simulink model "Simulation_cs_old"  (R2019a)
settings: Solver=ode5  StartTime=0.0  StopTime=inf  FixedStep=1/20  RelTol=1e-3
PreLoadFcn:
  | mbxruntime.callbacks.PreLoadFcn(bdroot);
PostLoadFcn:
  | mbxruntime.callbacks.PostLoadFcn(bdroot);
InitFcn:
  | mbxruntime.callbacks.InitFcn(bdroot);
StartFcn:
  | mbxruntime.callbacks.StartFcn(bdroot);
StopFcn:
  | mbxruntime.callbacks.StopFcn(bdroot);
model workspace: external: MAT-File .\Simulation_cs_hws.mat (data not in the file)
undefined symbols (not defined in the file or in its folder): DiscIntNeverNeededParam, InitImageOutputDir, mbxruntime, Simulation_cs_3ba1e87c6cdc7fd9, Simulation_cs_BMW_X5_SUV_1_Dynamics_Empty_STATE_BMW_X5_SUV_1_x0, Simulation_cs_BMW_X5_SUV_1_Dynamics_Empty_STATE_BMW_X5_SUV_1_y0, Simulation_cs_BMW_X5_SUV_1_Dynamics_Empty_STATE_BMW_X5_SUV_1_z0, Simulation_cs_dbe7801ee2d75073, Simulation_cs_f34d2d8469e03015
libraries: adeye_lib x45, robotlib x3, PreScanSimulinkLibrary x2, PreScanUsefulBlocks x1
(part 3 of 3)

== system Simulation_cs_old/PointCloudSensor_1 ==
  Sensor : S-Function  FunctionName=sfun_PCS  Parameters=mbxruntime.parameters.convert(sensorID), mbxruntime.parameters.convert(dataWidth), mbxruntime.parameters.convert(dataHeight), mbxruntime.parameters.convert(numChannels), mbxruntime.parameters.convert(dataType), mbxruntime.parameters.convert(timestep)  SFunctionDeploymentMode=off  EnableBusSupport=off  mask(PreScan Source Block: Point Cloud Sensor){sensorID=159, dataWidth=16, dataHeight=900, numChannels=4, dataType=0, timestep=1/20}
      mask prompts: sensorID "Sensor ID"; dataWidth "Data Width"; dataHeight "Data Height"; numChannels "Channel Count"; dataType "Data Type"; timestep "MATLAB timestep:"
      mask help: The Point Cloud Sensor provides XYZ positions relative to the sensor
      mask Help: eval('openHelp(6400)')
      mask Display: image(imread('PointCloudSensorSL.png'))
  PointCloudSensor_1 : Outport  Tag=outport/PointCloudInport  OutDataTypeStr=single  SampleTime=1/20
  wires:
  Sensor/1 -> PointCloudSensor_1/1

== system Simulation_cs_old/PointCloudSensor_2 ==
  Sensor : S-Function  FunctionName=sfun_PCS  Parameters=mbxruntime.parameters.convert(sensorID), mbxruntime.parameters.convert(dataWidth), mbxruntime.parameters.convert(dataHeight), mbxruntime.parameters.convert(numChannels), mbxruntime.parameters.convert(dataType), mbxruntime.parameters.convert(timestep)  SFunctionDeploymentMode=off  EnableBusSupport=off  mask(PreScan Source Block: Point Cloud Sensor){sensorID=160, dataWidth=16, dataHeight=900, numChannels=4, dataType=0, timestep=1/20}
      mask prompts: sensorID "Sensor ID"; dataWidth "Data Width"; dataHeight "Data Height"; numChannels "Channel Count"; dataType "Data Type"; timestep "MATLAB timestep:"
      mask help: The Point Cloud Sensor provides XYZ positions relative to the sensor
      mask Help: eval('openHelp(6400)')
      mask Display: image(imread('PointCloudSensorSL.png'))
  PointCloudSensor_2 : Outport  Tag=outport/PointCloudInport  OutDataTypeStr=single  SampleTime=1/20
  wires:
  Sensor/1 -> PointCloudSensor_2/1

== system Simulation_cs_old/PointCloudSensor_3 ==
  Sensor : S-Function  FunctionName=sfun_PCS  Parameters=mbxruntime.parameters.convert(sensorID), mbxruntime.parameters.convert(dataWidth), mbxruntime.parameters.convert(dataHeight), mbxruntime.parameters.convert(numChannels), mbxruntime.parameters.convert(dataType), mbxruntime.parameters.convert(timestep)  SFunctionDeploymentMode=off  EnableBusSupport=off  mask(PreScan Source Block: Point Cloud Sensor){sensorID=161, dataWidth=16, dataHeight=900, numChannels=4, dataType=0, timestep=1/20}
      mask prompts: sensorID "Sensor ID"; dataWidth "Data Width"; dataHeight "Data Height"; numChannels "Channel Count"; dataType "Data Type"; timestep "MATLAB timestep:"
      mask help: The Point Cloud Sensor provides XYZ positions relative to the sensor
      mask Help: eval('openHelp(6400)')
      mask Display: image(imread('PointCloudSensorSL.png'))
  PointCloudSensor_3 : Outport  Tag=outport/PointCloudInport  OutDataTypeStr=single  SampleTime=1/20
  wires:
  Sensor/1 -> PointCloudSensor_3/1

== system Simulation_cs_old/PointCloudSensor_4 ==
  Sensor : S-Function  FunctionName=sfun_PCS  Parameters=mbxruntime.parameters.convert(sensorID), mbxruntime.parameters.convert(dataWidth), mbxruntime.parameters.convert(dataHeight), mbxruntime.parameters.convert(numChannels), mbxruntime.parameters.convert(dataType), mbxruntime.parameters.convert(timestep)  SFunctionDeploymentMode=off  EnableBusSupport=off  mask(PreScan Source Block: Point Cloud Sensor){sensorID=162, dataWidth=16, dataHeight=900, numChannels=4, dataType=0, timestep=1/20}
      mask prompts: sensorID "Sensor ID"; dataWidth "Data Width"; dataHeight "Data Height"; numChannels "Channel Count"; dataType "Data Type"; timestep "MATLAB timestep:"
      mask help: The Point Cloud Sensor provides XYZ positions relative to the sensor
      mask Help: eval('openHelp(6400)')
      mask Display: image(imread('PointCloudSensorSL.png'))
  PointCloudSensor_4 : Outport  Tag=outport/PointCloudInport  OutDataTypeStr=single  SampleTime=1/20
  wires:
  Sensor/1 -> PointCloudSensor_4/1

== system Simulation_cs_old/PreScanTerminator ==
  Terminator : Terminator
  sfun_Terminator : S-Function  FunctionName=sfun_Terminator  Parameters=SampleTime  SFunctionDeploymentMode=off  EnableBusSupport=off  mask(Legacy Function){SFunctionSpec=void prescan_terminator_outputFcn(void ** work1, PRESCAN_TERMINATORDATA y1[1]), SampleTime=TimeStep, ShowSpec=on}
      mask prompts: SampleTime "Sample time (-1 for inherited):"; ShowSpec "Display function specification"
      mask help:
      | This block allows you to call the legacy functions specified by the following Legacy Code Tool definition:
      | def.SFunctionName = 'sfun_Terminator';
      | def.OutputFcnSpec = 'void prescan_terminator_outputFcn(void ** work1, PRESCAN_TERMINATORDATA y1[1])';
      | def.StartFcnSpec = 'void prescan_terminator_startFcn(void ** work1)';
      | def.TerminateFcnSpec = 'void prescan_terminator_terminateFcn(void ** work1)';
      | def.HeaderFiles = {'prescan_terminator_data.h'};
      | def.HostLibFiles = {'sensorinterfaced.lib'};
      | def.IncPaths = {'src', 'C:\prescandev\vislibrary\vis\..\pimp\include\sensors\InterfaceRTW'};
      | def.SrcPaths = {'src'};
      | def.LibPaths = {'C:\\prescandev\\vislibrary_build\lib'};
      | def.SampleTime = 'parameterized';
      | def.Options.language = 'C';
      mask Help: <p>This block was generated automatically by the Legacy Code Tool. For detailed help on this tool, call<a href="matlab:legacy_code('help')"> legacy_code('help')</a>.</p>
      mask Callback ShowSpec:
      | if strcmp(get_param(gcbh, 'ShowSpec'), 'on')
      |   set_param(gcbh, 'MaskDisplay', sprintf('fprintf(''%s'');', get_param(gcbh, 'SFunctionSpec')));
      | else
      |   set_param(gcbh, 'MaskDisplay', sprintf('fprintf(''%s'');', get_param(gcbh, 'FunctionName')));
      | end
      mask Display: fprintf('void prescan_terminator_outputFcn(void ** work1, PRESCAN_TERMINATORDATA y1[1])');
  wires:
  sfun_Terminator/1 -> Terminator/1

== system Simulation_cs_old/Radar_1 ==
  Sensor : S-Function  FunctionName=sfun_Radar  Parameters=mbxruntime.parameters.convert(sensorID), mbxruntime.parameters.convert(detectableObjects), mbxruntime.parameters.convert(timestep)  SFunctionDeploymentMode=off  EnableBusSupport=off  mask(PreScan Source Block: Radar Sensor){sensorID=165, detectableObjects=7, timestep=1/20}
      mask prompts: sensorID "Sensor ID"; detectableObjects "Max detectable objects:"; timestep "MATLAB timestep:"
      mask help:
      | The Radar Sensor is a detailed sensor based on a physical radar
      | model that includes Antenna GAIN Maps (AGM) and atmospheric
      | attenuation.
      |
      | For more information, please click Help.
      mask Help: eval('openHelp(1464)')
      mask Display: image(imread('Radar.png'))
  Radar_1 : Outport  Tag=outport/Radar  OutDataTypeStr=Bus: PRESCAN_SCANNERSENSOR_MESSAGE  PortDimensions=7  SampleTime=1/20
  wires:
  Sensor/1 -> Radar_1/1

== system Simulation_cs_old/SELF_BMW_X5_SUV_1 ==
  Sensor : S-Function  FunctionName=sfun_SelfSensor  Parameters=mbxruntime.parameters.convert(UniqueID), mbxruntime.parameters.convert(TimeStep)  SFunctionDeploymentMode=off  EnableBusSupport=off  mask(PreScan Source Block: SELF){UniqueID=158, TimeStep=1/20}
      mask prompts: UniqueID "Auto-Assigned: Unique ID"; TimeStep "Auto-Assigned: Upload Period [s]"
      mask help:
      | The SELF port shows (state) information of the actor itself. The outputs are position in the experiment's axis system and the GPS coordinates, and the object's absolute velocity and compass heading.
      |
      | For more information, please click Help.
      mask Help: eval('openHelp(462)')
      mask Display: image(imread('GPS.png'))
  SELF_BMW_X5_SUV_1 : Outport  Tag=outport/SelfPort  OutDataTypeStr=Bus: PRESCAN_SELFSENSORDATA  PortDimensions=1  SampleTime=1/20
  wires:
  Sensor/1 -> SELF_BMW_X5_SUV_1/1

== system Simulation_cs_old/STATE_BMW_X5_SUV_1_bus ==
  STATE_BMW_X5_SUV_1_bus : Inport  Tag=inport/StatePort  OutDataTypeStr=Bus: PRESCAN_STATEACTUATORDATA  PortDimensions=1  SampleTime=1/20  BusOutputAsStruct=on
  Actuator : S-Function  FunctionName=sfun_StateActuator  Parameters=mbxruntime.parameters.convert(UniqueID), mbxruntime.parameters.convert(TimeStep)  SFunctionDeploymentMode=off  EnableBusSupport=off  mask(PreScan Sink Block: State){UniqueID=158, TimeStep=1/20}
      mask prompts: UniqueID "Auto-Assigned: Unique ID"; TimeStep "Auto-Assigned: Upload Period [s]"
      mask help:
      | The Actor State contains a vector signal of size (9x1), containing the following signals:
      |
      | -  Position    	(x,y,z)             	[m]
      | -  Velocity    	(vx,vy,vz)         	[m/s]
      | -  Angles       	(Roll, Pitch, Yaw)	[rad]
      |
      | The Actor state is defined in the global axis system.
      | The state is superponed on the Initial position defined in the GUI.
      |
      | For more information, please click Help.
      mask Help: eval('openHelp(222)')
      mask Display: image(imread('State.png'))
  wires:
  STATE_BMW_X5_SUV_1_bus/1 -> Actuator/1

== system Simulation_cs_old/ScenarioEngine ==
  Clock : Clock
  sfun_ScenarioEngine : S-Function  FunctionName=sfun_ScenarioEngine  Parameters=TimeStep  SFunctionDeploymentMode=off  EnableBusSupport=off
  wires:
  Clock/1 -> sfun_ScenarioEngine/1

== system Simulation_cs_old/Synchronizer ==
  Bus Selector1 : BusSelector  OutputSignals=FederateStopped
  Stop Simulation : Stop
  sfun_Synchronizer : S-Function  FunctionName=sfun_Synchronizer  Parameters=SampleTime  SFunctionDeploymentMode=off  EnableBusSupport=off  mask(Legacy Function){SFunctionSpec=void prescan_synchronizer_outputFcn(void ** work1, PRESCAN_SYNCHRONIZEDATA y1[1]), SampleTime=TimeStep, ShowSpec=on}
      mask prompts: SampleTime "Sample time (-1 for inherited):"; ShowSpec "Display function specification"
      mask help:
      | This block allows you to call the legacy functions specified by the following Legacy Code Tool definition:
      | def.SFunctionName = 'sfun_Synchronizer';
      | def.OutputFcnSpec = 'void prescan_synchronizer_outputFcn(void ** work1, PRESCAN_TIMESTAMPDATA u1[1], PRESCAN_SYNCHRONIZEDATA y1[1])';
      | def.StartFcnSpec = 'void prescan_synchronizer_startFcn(void ** work1)';
      | def.TerminateFcnSpec = 'void prescan_synchronizer_terminateFcn(void ** work1)';
      | def.HeaderFiles = {'prescan_synchronizer_data.h'};
      | def.HostLibFiles = {'sensorinterfaced.lib'};
      | def.IncPaths = {'src', 'C:\prescandev\vislibrary\vis\..\pimp\include\sensors\InterfaceRTW'};
      | def.SrcPaths = {'src'};
      | def.LibPaths = {'C:\\prescandev\\vislibrary_build\lib'};
      | def.SampleTime = 'parameterized';
      | def.Options.language = 'C';
      mask Help: <p>This block was generated automatically by the Legacy Code Tool. For detailed help on this tool, call<a href="matlab:legacy_code('help')"> legacy_code('help')</a>.</p>
      mask Callback ShowSpec:
      | if strcmp(get_param(gcbh, 'ShowSpec'), 'on')
      |   set_param(gcbh, 'MaskDisplay', sprintf('fprintf(''%s'');', get_param(gcbh, 'SFunctionSpec')));
      | else
      |   set_param(gcbh, 'MaskDisplay', sprintf('fprintf(''%s'');', get_param(gcbh, 'FunctionName')));
      | end
      mask Display: fprintf('void prescan_synchronizer_outputFcn(void ** work1, PRESCAN_SYNCHRONIZEDATA y1[1])');
  wires:
  sfun_Synchronizer/1 -> Bus Selector1/1
  Bus Selector1/1 -> Stop Simulation/1  "<FederateStopped>"

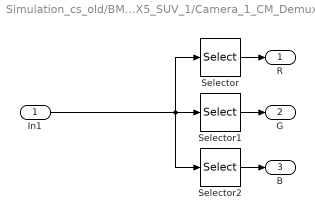
== system Simulation_cs_old/BMW_X5_SUV_1/Camera_1_CM_Demux ==
  In1 : Inport
  Selector : Selector  NumberOfDimensions=2  InputPortWidth=3  IndexOptions=Index vector (dialog),Index vector (dialog)  Indices=-1,1:hres  OutputSizes=1,1
  Selector1 : Selector  NumberOfDimensions=2  InputPortWidth=3  IndexOptions=Index vector (dialog),Index vector (dialog)  Indices=-1,hres+1:hres*2  OutputSizes=1,1
  Selector2 : Selector  NumberOfDimensions=2  InputPortWidth=3  IndexOptions=Index vector (dialog),Index vector (dialog)  Indices=-1,hres*2+1:hres*3  OutputSizes=1,1
  R : Outport
  G : Outport  Port=2
  B : Outport  Port=3
  wires:
  In1/1 -> Selector1/1, Selector/1, Selector2/1
  Selector/1 -> R/1
  Selector1/1 -> G/1
  Selector2/1 -> B/1

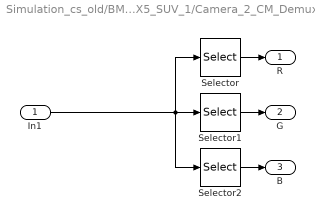
== system Simulation_cs_old/BMW_X5_SUV_1/Camera_2_CM_Demux ==
  In1 : Inport
  Selector : Selector  NumberOfDimensions=2  InputPortWidth=3  IndexOptions=Index vector (dialog),Index vector (dialog)  Indices=-1,1:hres  OutputSizes=1,1
  Selector1 : Selector  NumberOfDimensions=2  InputPortWidth=3  IndexOptions=Index vector (dialog),Index vector (dialog)  Indices=-1,hres+1:hres*2  OutputSizes=1,1
  Selector2 : Selector  NumberOfDimensions=2  InputPortWidth=3  IndexOptions=Index vector (dialog),Index vector (dialog)  Indices=-1,hres*2+1:hres*3  OutputSizes=1,1
  R : Outport
  G : Outport  Port=2
  B : Outport  Port=3
  wires:
  In1/1 -> Selector1/1, Selector/1, Selector2/1
  Selector/1 -> R/1
  Selector1/1 -> G/1
  Selector2/1 -> B/1

== system Simulation_cs_old/BMW_X5_SUV_1/Camera_tl_CM_Demux ==
  In1 : Inport
  Selector : Selector  NumberOfDimensions=2  InputPortWidth=3  IndexOptions=Index vector (dialog),Index vector (dialog)  Indices=-1,1:hres  OutputSizes=1,1
  Selector1 : Selector  NumberOfDimensions=2  InputPortWidth=3  IndexOptions=Index vector (dialog),Index vector (dialog)  Indices=-1,hres+1:hres*2  OutputSizes=1,1
  Selector2 : Selector  NumberOfDimensions=2  InputPortWidth=3  IndexOptions=Index vector (dialog),Index vector (dialog)  Indices=-1,hres*2+1:hres*3  OutputSizes=1,1
  R : Outport
  G : Outport  Port=2
  B : Outport  Port=3
  wires:
  In1/1 -> Selector1/1, Selector/1, Selector2/1
  Selector/1 -> R/1
  Selector1/1 -> G/1
  Selector2/1 -> B/1

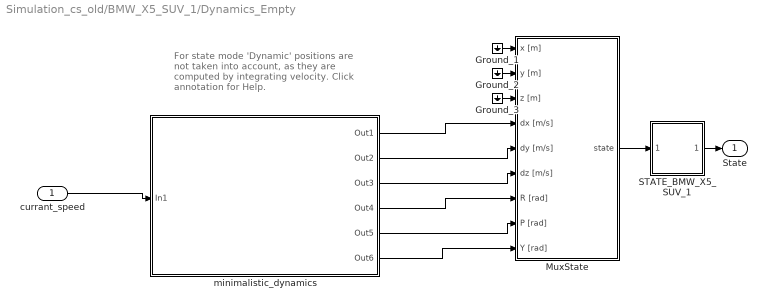
== system Simulation_cs_old/BMW_X5_SUV_1/Dynamics_Empty ==
  note: For state mode 'Dynamic' positions
      | are not taken into account, as they
      | are computed by integrating velocity.
      | Click annotation for Help.
  currant_speed : Inport
  Ground_1 : Ground
  Ground_2 : Ground
  Ground_3 : Ground
  MuxState : Subsystem  Tag=mux/State  mask(Empty Dynamics State Block){positioningmode=off, TimeStep=1/20}
      mask prompts: positioningmode "Positioning Mode"; TimeStep "Auto Assigned: Time Step [s]"
      mask help:
      | Build the state of an actor based on user input.
      | The user can either use positioning mode or dynamics mode.
      | - When using positioning mode the position and orientation of the actor are set directly based on the input. Expected input is relative to the initial position and orientation of the actor. It's also possible to specify the velocity of the actor, though this input isn't used, only passed on.
      | - When using dynamics mode the position input is ignored. Expected input is velocity and orientation. The velocity is relative the current orientation of the actor, while orientation is relative to its initial orientation. The position of the actor is calculated based on the velocity and orientation given.
      settings: DeleteFcn=PreScanBlockDeleteFcn;
  STATE_BMW_X5_SUV_1 : Subsystem  Tag=mux/StatePort  Priority=0  LoadFcn=load PrescanStateActuatorData  mask(PreScan Sink Block: State){x0=Simulation_cs_BMW_X5_SUV_1_Dynamics_Empty_STATE_BMW_X5_SUV_1_x0, y0=Simulation_cs_BMW_X5_SUV_1_Dynamics_Empty_STATE_BMW_X5_SUV_1_y0, z0=Simulation_cs_BMW_X5_SUV_1_Dynamics_Empty_STATE_BMW_X5_SUV_1_z0, Roll0=Simulation_cs_dbe7801ee2d75073, Pitch0=Simulation_cs_3ba1e87c6cdc7fd9, Yaw0=Simulation_cs_f34d2d8469e03015, TimeStep=1/20}
      mask prompts: x0 "Ini x-position VEHICLE wrt GLOBAL axis system [m]"; y0 "Ini y-position VEHICLE wrt GLOBAL axis system [m]"; z0 "Ini z-position VEHICLE wrt GLOBAL axis system [m]"; Roll0 "Ini roll-angle BODY wrt VEHICLE axis system [deg]"; Pitch0 "Ini pitch-angle BODY wrt VEHICLE axis system [deg]"; Yaw0 "Ini yaw-angle VEHICLE wrt GLOBAL axis system [deg]"; TimeStep "Auto-Assigned: Upload Period [s]"
      mask help:
      | The Actor State contains a vector signal of size (9x1), containing the following signals:
      |
      | -  Position                  (x,y,z)                                     [m]
      | -  Velocity                  (vx,vy,vz)                               [m/s]
      | -  Angles                    (Roll, Pitch, Yaw)                   [rad]
      |
      | The Actor state is defined in the global axis system.
      | The state is superponed on the Initial position defined in the GUI.
      |
      | For more information, please click Help.
      settings: DeleteFcn=PreScanBlockDeleteFcn;
      mask Help: eval('openHelp(222)')
      mask Display: image(imread('State.png'))
  minimalistic_dynamics : Subsystem  AncestorBlock=adeye_lib/minimalistic_dynamics
      mask Display:
      | fprintf('Minimalistic Dynamics\n\n')
      | 
      | port_label('input',1,'velocity[m/s]')
      | 
      | port_label('output',1,'dx [m/s]')
      | port_label('output',2,'dy [m/s]')
      | port_label('output',3,'dz [m/s]')
      | port_label('output',4,'R [rad]')
      | port_label('output',5,'P [rad]')
      | port_label('output',6,'Y [rad]')
  State : Outport  Tag=outport/StateOutport  SampleTime=1/20
  wires:
  minimalistic_dynamics/1(Out1) -> MuxState/4(dx [m/s])
  minimalistic_dynamics/2(Out2) -> MuxState/5(dy [m/s])
  minimalistic_dynamics/3(Out3) -> MuxState/6(dz [m/s])
  minimalistic_dynamics/4(Out4) -> MuxState/7(R [rad])
  minimalistic_dynamics/5(Out5) -> MuxState/8(P [rad])
  minimalistic_dynamics/6(Out6) -> MuxState/9(Y [rad])
  currant_speed/1 -> minimalistic_dynamics/1(In1)
  MuxState/1(state) -> STATE_BMW_X5_SUV_1/1(State)
  STATE_BMW_X5_SUV_1/1(StateBus) -> State/1
  Ground_1/1 -> MuxState/1(x [m])
  Ground_2/1 -> MuxState/2(y [m])
  Ground_3/1 -> MuxState/3(z [m])

== system Simulation_cs_old/BMW_X5_SUV_1/PointCloudSensor_1_Angles_Demux ==
  In2 : Inport
  Selector : Selector  NumberOfDimensions=2  InputPortWidth=3  IndexOptions=Index vector (dialog),Index vector (dialog)  Indices=-1,offset+1:(offset+hres)  OutputSizes=1,1
  Selector1 : Selector  NumberOfDimensions=2  InputPortWidth=3  IndexOptions=Index vector (dialog),Index vector (dialog)  Indices=-1,(offset+hres+1):(offset+2*hres)  OutputSizes=1,1
  Theta : Outport
  Phi : Outport  Port=2
  wires:
  Selector1/1 -> Phi/1
  Selector/1 -> Theta/1
  In2/1 -> Selector/1, Selector1/1

== system Simulation_cs_old/BMW_X5_SUV_1/PointCloudSensor_1_Intensity_Demux ==
  In1 : Inport
  Selector3 : Selector  NumberOfDimensions=2  InputPortWidth=3  IndexOptions=Index vector (dialog),Index vector (dialog)  Indices=-1,offset+1:(offset+hres)  OutputSizes=1,1
  Intensity : Outport
  wires:
  Selector3/1 -> Intensity/1
  In1/1 -> Selector3/1

== system Simulation_cs_old/BMW_X5_SUV_1/PointCloudSensor_1_Range_Demux ==
  In1 : Inport
  Selector : Selector  NumberOfDimensions=2  InputPortWidth=3  IndexOptions=Index vector (dialog),Index vector (dialog)  Indices=-1,offset+1:(offset+hres)  OutputSizes=1,1
  Range : Outport
  wires:
  Selector/1 -> Range/1
  In1/1 -> Selector/1

== system Simulation_cs_old/BMW_X5_SUV_1/PointCloudSensor_2_Angles_Demux ==
  In2 : Inport
  Selector : Selector  NumberOfDimensions=2  InputPortWidth=3  IndexOptions=Index vector (dialog),Index vector (dialog)  Indices=-1,offset+1:(offset+hres)  OutputSizes=1,1
  Selector1 : Selector  NumberOfDimensions=2  InputPortWidth=3  IndexOptions=Index vector (dialog),Index vector (dialog)  Indices=-1,(offset+hres+1):(offset+2*hres)  OutputSizes=1,1
  Theta : Outport
  Phi : Outport  Port=2
  wires:
  Selector1/1 -> Phi/1
  Selector/1 -> Theta/1
  In2/1 -> Selector/1, Selector1/1

== system Simulation_cs_old/BMW_X5_SUV_1/PointCloudSensor_2_Intensity_Demux ==
  In1 : Inport
  Selector3 : Selector  NumberOfDimensions=2  InputPortWidth=3  IndexOptions=Index vector (dialog),Index vector (dialog)  Indices=-1,offset+1:(offset+hres)  OutputSizes=1,1
  Intensity : Outport
  wires:
  Selector3/1 -> Intensity/1
  In1/1 -> Selector3/1

== system Simulation_cs_old/BMW_X5_SUV_1/PointCloudSensor_2_Range_Demux ==
  In1 : Inport
  Selector : Selector  NumberOfDimensions=2  InputPortWidth=3  IndexOptions=Index vector (dialog),Index vector (dialog)  Indices=-1,offset+1:(offset+hres)  OutputSizes=1,1
  Range : Outport
  wires:
  Selector/1 -> Range/1
  In1/1 -> Selector/1

== system Simulation_cs_old/BMW_X5_SUV_1/PointCloudSensor_3_Angles_Demux ==
  In2 : Inport
  Selector : Selector  NumberOfDimensions=2  InputPortWidth=3  IndexOptions=Index vector (dialog),Index vector (dialog)  Indices=-1,offset+1:(offset+hres)  OutputSizes=1,1
  Selector1 : Selector  NumberOfDimensions=2  InputPortWidth=3  IndexOptions=Index vector (dialog),Index vector (dialog)  Indices=-1,(offset+hres+1):(offset+2*hres)  OutputSizes=1,1
  Theta : Outport
  Phi : Outport  Port=2
  wires:
  Selector1/1 -> Phi/1
  Selector/1 -> Theta/1
  In2/1 -> Selector/1, Selector1/1

== system Simulation_cs_old/BMW_X5_SUV_1/PointCloudSensor_3_Intensity_Demux ==
  In1 : Inport
  Selector3 : Selector  NumberOfDimensions=2  InputPortWidth=3  IndexOptions=Index vector (dialog),Index vector (dialog)  Indices=-1,offset+1:(offset+hres)  OutputSizes=1,1
  Intensity : Outport
  wires:
  Selector3/1 -> Intensity/1
  In1/1 -> Selector3/1

== system Simulation_cs_old/BMW_X5_SUV_1/PointCloudSensor_3_Range_Demux ==
  In1 : Inport
  Selector : Selector  NumberOfDimensions=2  InputPortWidth=3  IndexOptions=Index vector (dialog),Index vector (dialog)  Indices=-1,offset+1:(offset+hres)  OutputSizes=1,1
  Range : Outport
  wires:
  Selector/1 -> Range/1
  In1/1 -> Selector/1

== system Simulation_cs_old/BMW_X5_SUV_1/PointCloudSensor_4_Angles_Demux ==
  In2 : Inport
  Selector : Selector  NumberOfDimensions=2  InputPortWidth=3  IndexOptions=Index vector (dialog),Index vector (dialog)  Indices=-1,offset+1:(offset+hres)  OutputSizes=1,1
  Selector1 : Selector  NumberOfDimensions=2  InputPortWidth=3  IndexOptions=Index vector (dialog),Index vector (dialog)  Indices=-1,(offset+hres+1):(offset+2*hres)  OutputSizes=1,1
  Theta : Outport
  Phi : Outport  Port=2
  wires:
  Selector1/1 -> Phi/1
  Selector/1 -> Theta/1
  In2/1 -> Selector/1, Selector1/1

== system Simulation_cs_old/BMW_X5_SUV_1/PointCloudSensor_4_Intensity_Demux ==
  In1 : Inport
  Selector3 : Selector  NumberOfDimensions=2  InputPortWidth=3  IndexOptions=Index vector (dialog),Index vector (dialog)  Indices=-1,offset+1:(offset+hres)  OutputSizes=1,1
  Intensity : Outport
  wires:
  Selector3/1 -> Intensity/1
  In1/1 -> Selector3/1

== system Simulation_cs_old/BMW_X5_SUV_1/PointCloudSensor_4_Range_Demux ==
  In1 : Inport
  Selector : Selector  NumberOfDimensions=2  InputPortWidth=3  IndexOptions=Index vector (dialog),Index vector (dialog)  Indices=-1,offset+1:(offset+hres)  OutputSizes=1,1
  Range : Outport
  wires:
  Selector/1 -> Range/1
  In1/1 -> Selector/1

== system Simulation_cs_old/BMW_X5_SUV_1/Radar_1_Demux ==
  Radar : Inport
  Bus Selector1 : BusSelector  OutputSignals=ActiveBeamID[-],Range[m],DopplerVelocity[ms-1],DopplerVelocityX[ms-1],DopplerVelocityY[ms-1],DopplerVelocityZ[ms-1],Theta[deg],Phi[deg],TargetID[-],TargetTypeID[-],EnergyLoss[dB],Alpha[deg],Beta[deg]  OutputAsBus=on
  ScannerSensorLegacyBusConversion : PreScanUsefulBlocks/ScannerSensorLegacyBusConversion  MAXMESSAGES=MAXMESSAGES
  Radar Data : Outport
  Timestamp : Outport  Port=2
  wires:
  ScannerSensorLegacyBusConversion/2 -> Timestamp/1
  Bus Selector1/1 -> Radar Data/1
  ScannerSensorLegacyBusConversion/1 -> Bus Selector1/1
  Radar/1 -> ScannerSensorLegacyBusConversion/1

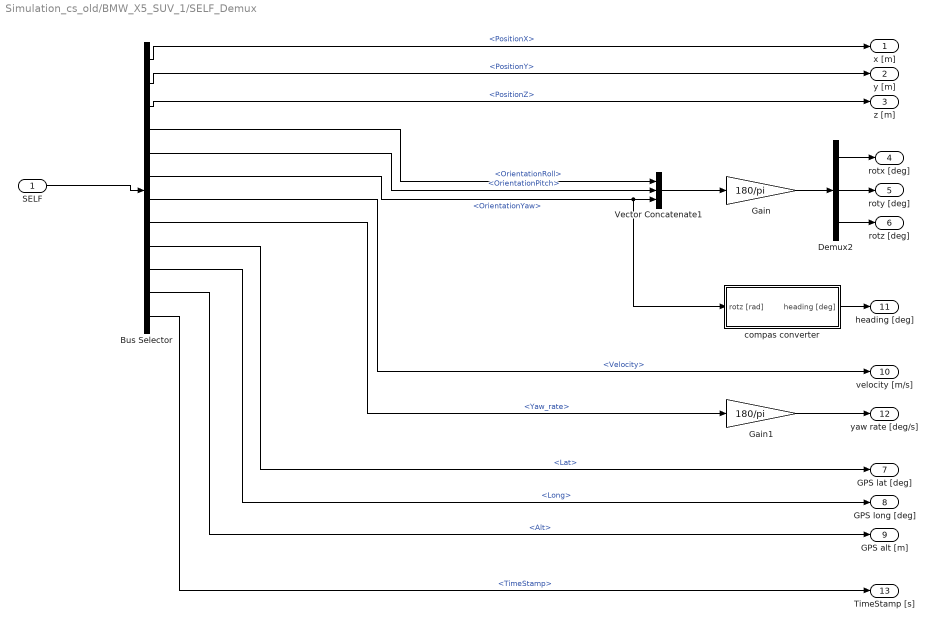
== system Simulation_cs_old/BMW_X5_SUV_1/SELF_Demux ==
  SELF : Inport  OutDataTypeStr=Bus: PRESCAN_SELFSENSORDATA
  Bus Selector : BusSelector  OutputSignals=PositionX,PositionY,PositionZ,OrientationRoll,OrientationPitch,OrientationYaw,Velocity,Yaw_rate,Lat,Long,Alt,TimeStamp
  Demux2 : Demux  Outputs=3
  Gain : Gain  Gain=180/pi
  Gain1 : Gain  Gain=180/pi
  Vector Concatenate1 : Concatenate  NumInputs=3
  compas converter : Subsystem
  x [m] : Outport
  y [m] : Outport  Port=2
  z [m] : Outport  Port=3
  rotx [deg] : Outport  Port=4
  roty [deg] : Outport  Port=5
  rotz [deg] : Outport  Port=6
  GPS lat [deg] : Outport  Port=7
  GPS long [deg] : Outport  Port=8
  GPS alt [m] : Outport  Port=9
  velocity [m/s] : Outport  Port=10
  heading [deg] : Outport  Port=11
  yaw rate [deg/s] : Outport  Port=12
  TimeStamp [s] : Outport  Port=13
  wires:
  Bus Selector/12 -> TimeStamp [s]/1  "<TimeStamp>"
  Bus Selector/11 -> GPS alt [m]/1  "<Alt>"
  Bus Selector/10 -> GPS long [deg]/1  "<Long>"
  Bus Selector/9 -> GPS lat [deg]/1  "<Lat>"
  Bus Selector/8 -> Gain1/1  "<Yaw_rate>"
  Bus Selector/7 -> velocity [m/s]/1  "<Velocity>"
  Bus Selector/6 -> compas converter/1(rotz [rad]), Vector Concatenate1/3  "<OrientationYaw>"
  Bus Selector/5 -> Vector Concatenate1/2  "<OrientationPitch>"
  Bus Selector/4 -> Vector Concatenate1/1  "<OrientationRoll>"
  Vector Concatenate1/1 -> Gain/1
  Bus Selector/3 -> z [m]/1  "<PositionZ>"
  Bus Selector/2 -> y [m]/1  "<PositionY>"
  Bus Selector/1 -> x [m]/1  "<PositionX>"
  SELF/1 -> Bus Selector/1
  Gain/1 -> Demux2/1
  Demux2/1 -> rotx [deg]/1
  Demux2/2 -> roty [deg]/1
  Demux2/3 -> rotz [deg]/1
  compas converter/1(heading [deg]) -> heading [deg]/1
  Gain1/1 -> yaw rate [deg/s]/1

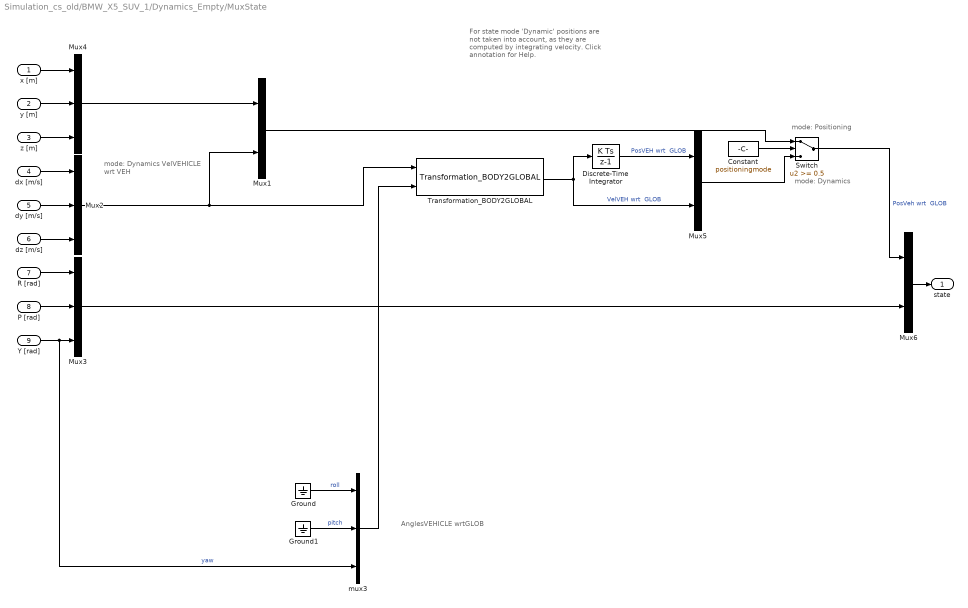
== system Simulation_cs_old/BMW_X5_SUV_1/Dynamics_Empty/MuxState ==
  note: mode: Dynamics
  note: mode: Positioning
  note: mode: Dynamics
      | VelVEHICLE
      | wrt VEH
  note: AnglesVEHICLE
      | wrtGLOB
  note: For state mode 'Dynamic' positions
      | are not taken into account, as they
      | are computed by integrating velocity.
      | Click annotation for Help.
  x [m] : Inport  SampleTime=TimeStep
  y [m] : Inport  Port=2  SampleTime=TimeStep
  z [m] : Inport  Port=3  SampleTime=TimeStep
  dx [m/s] : Inport  Port=4  SampleTime=TimeStep
  dy [m/s] : Inport  Port=5  SampleTime=TimeStep
  dz [m/s] : Inport  Port=6  SampleTime=TimeStep
  R [rad] : Inport  Port=7  SampleTime=TimeStep
  P [rad] : Inport  Port=8  SampleTime=TimeStep
  Y [rad] : Inport  Port=9  SampleTime=TimeStep
  Constant : Constant  DisableCoverage=on  Value=positioningmode
  Discrete-Time Integrator : DiscreteIntegrator  SampleTime=TimeStep  ICPrevOutput=DiscIntNeverNeededParam  ICPrevScaledInput=DiscIntNeverNeededParam
  Ground : Ground
  Ground1 : Ground
  Mux1 : Mux  Inputs=[3 3]
  Mux2 : Mux  Inputs=3
  Mux3 : Mux  Inputs=3
  Mux4 : Mux  Inputs=3
  Mux5 : Mux  Inputs=[3 3]
  Mux6 : Mux  Inputs=[6 3]
  Switch : Switch  Threshold=0.5
  Transformation_BODY2GLOBAL : PreScanSimulinkLibrary/Simple_Vehicle_Dynamics/Chassis/MuxDynState/Transformation_BODY2GLOBAL  SystemSampleTime=-1
  mux3 : Mux  Inputs=3
  state : Outport
  wires:
  Constant/1 -> Switch/2
  Mux6/1 -> state/1
  Mux4/1 -> Mux1/1
  Mux5/1 -> Switch/3
  Mux1/1 -> Switch/1
  Switch/1 -> Mux6/1  "PosVeh wrt  GLOB"
  P [rad]/1 -> Mux3/2
  R [rad]/1 -> Mux3/1
  dz [m/s]/1 -> Mux2/3
  dy [m/s]/1 -> Mux2/2
  dx [m/s]/1 -> Mux2/1
  z [m]/1 -> Mux4/3
  y [m]/1 -> Mux4/2
  x [m]/1 -> Mux4/1
  Ground1/1 -> mux3/2  "pitch"
  Y [rad]/1 -> mux3/3, Mux3/3  "yaw"
  Mux3/1 -> Mux6/2
  Transformation_BODY2GLOBAL/1 -> Discrete-Time Integrator/1, Mux5/2  "VelVEH wrt  GLOB"
  mux3/1 -> Transformation_BODY2GLOBAL/2
  Ground/1 -> mux3/1  "roll"
  Mux2/1 -> Mux1/2, Transformation_BODY2GLOBAL/1
  Discrete-Time Integrator/1 -> Mux5/1  "PosVEH wrt  GLOB"

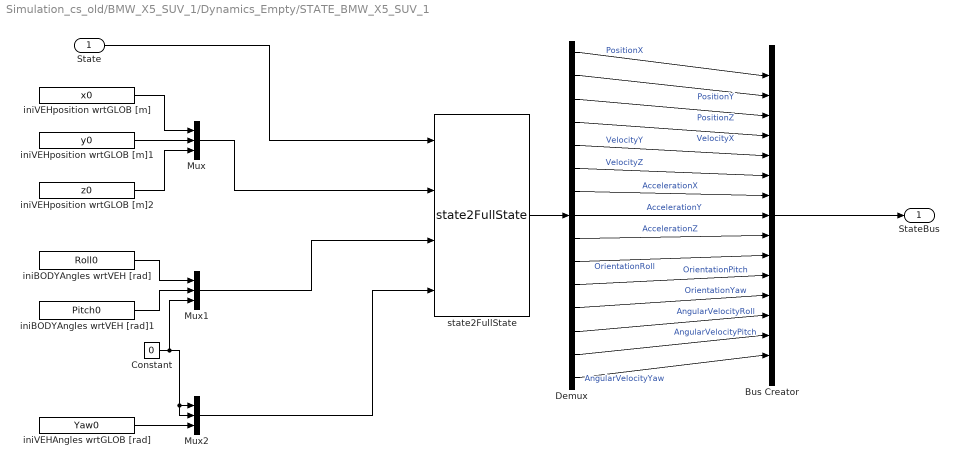
== system Simulation_cs_old/BMW_X5_SUV_1/Dynamics_Empty/STATE_BMW_X5_SUV_1 ==
  State : Inport  SampleTime=TimeStep
  Bus Creator : BusCreator  Inputs=15  OutDataTypeStr=Bus: PRESCAN_STATEACTUATORDATA  NonVirtualBus=on
  Constant : Constant  Value=0
  Demux : Demux  Outputs=15
  Mux : Mux  Inputs=3
  Mux1 : Mux  Inputs=3
  Mux2 : Mux  Inputs=3
  iniBODYAngles wrtVEH [rad] : Constant  Value=Roll0  SampleTime=TimeStep
  iniBODYAngles wrtVEH [rad]1 : Constant  Value=Pitch0  SampleTime=TimeStep
  iniVEHAngles wrtGLOB [rad] : Constant  Value=Yaw0  SampleTime=TimeStep
  iniVEHposition wrtGLOB [m] : Constant  Value=x0  SampleTime=TimeStep
  iniVEHposition wrtGLOB [m]1 : Constant  Value=y0  SampleTime=TimeStep
  iniVEHposition wrtGLOB [m]2 : Constant  Value=z0  SampleTime=TimeStep
  state2FullState : PreScanSimulinkLibrary/state2FullState  SystemSampleTime=-1
  StateBus : Outport  OutDataTypeStr=Bus: PRESCAN_STATEACTUATORDATA
  wires:
  Mux2/1 -> state2FullState/4
  iniVEHAngles wrtGLOB [rad]/1 -> Mux2/3
  Mux1/1 -> state2FullState/3
  Constant/1 -> Mux2/1, Mux2/2, Mux1/3
  iniBODYAngles wrtVEH [rad]1/1 -> Mux1/2
  iniBODYAngles wrtVEH [rad]/1 -> Mux1/1
  Mux/1 -> state2FullState/2
  iniVEHposition wrtGLOB [m]2/1 -> Mux/3
  iniVEHposition wrtGLOB [m]/1 -> Mux/1
  iniVEHposition wrtGLOB [m]1/1 -> Mux/2
  Demux/15 -> Bus Creator/15  "AngularVelocityYaw"
  Demux/14 -> Bus Creator/14  "AngularVelocityPitch"
  Demux/13 -> Bus Creator/13  "AngularVelocityRoll"
  Demux/12 -> Bus Creator/12  "OrientationYaw"
  Demux/11 -> Bus Creator/11  "OrientationPitch"
  Demux/10 -> Bus Creator/10  "OrientationRoll"
  Demux/9 -> Bus Creator/9  "AccelerationZ"
  Demux/8 -> Bus Creator/8  "AccelerationY"
  Demux/7 -> Bus Creator/7  "AccelerationX"
  Demux/6 -> Bus Creator/6  "VelocityZ"
  Demux/5 -> Bus Creator/5  "VelocityY"
  Demux/4 -> Bus Creator/4  "VelocityX"
  Demux/3 -> Bus Creator/3  "PositionZ"
  Demux/2 -> Bus Creator/2  "PositionY"
  Demux/1 -> Bus Creator/1  "PositionX"
  state2FullState/1 -> Demux/1
  State/1 -> state2FullState/1
  Bus Creator/1 -> StateBus/1

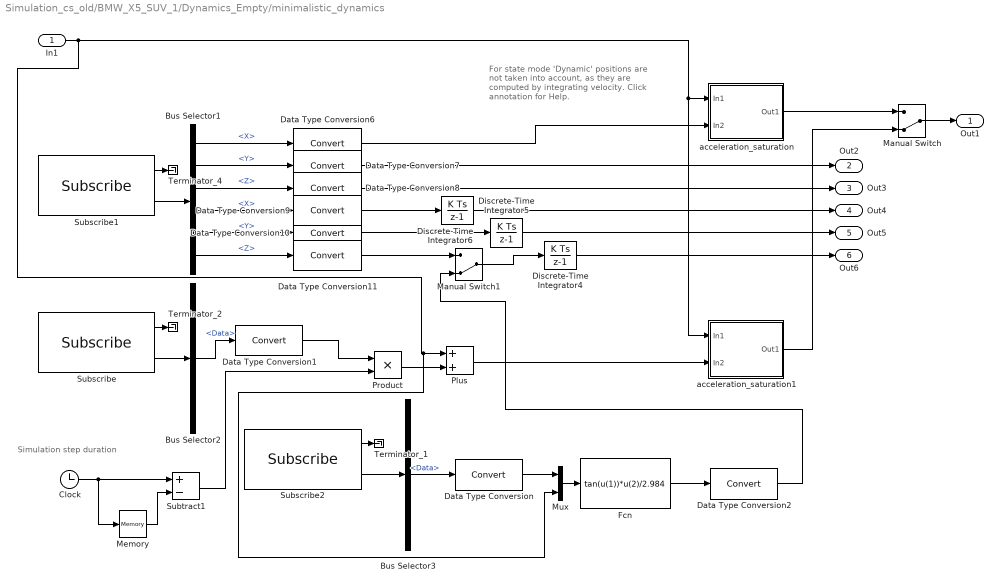
== system Simulation_cs_old/BMW_X5_SUV_1/Dynamics_Empty/minimalistic_dynamics ==
  note: For state mode 'Dynamic' positions
      | are not taken into account, as they
      | are computed by integrating velocity.
      | Click annotation for Help.
  note: Simulation step duration
  In1 : Inport
  Bus Selector1 : BusSelector  OutputSignals=Twist.Linear.X,Twist.Linear.Y,Twist.Linear.Z,Twist.Angular.X,Twist.Angular.Y,Twist.Angular.Z
  Bus Selector2 : BusSelector  OutputSignals=Data
  Bus Selector3 : BusSelector  OutputSignals=Data
  Clock : Clock
  Data Type Conversion{,1..2,6..11} (9 alike) : DataTypeConversion
  Discrete-Time Integrator4 : DiscreteIntegrator  SampleTime=-1  ICPrevOutput=DiscIntNeverNeededParam  ICPrevScaledInput=DiscIntNeverNeededParam
  Discrete-Time Integrator5 : DiscreteIntegrator  SampleTime=-1  ICPrevOutput=DiscIntNeverNeededParam  ICPrevScaledInput=DiscIntNeverNeededParam
  Discrete-Time Integrator6 : DiscreteIntegrator  SampleTime=-1  ICPrevOutput=DiscIntNeverNeededParam  ICPrevScaledInput=DiscIntNeverNeededParam
  Fcn : Fcn  Expr=tan(u(1))*u(2)/2.984
  Manual Switch : ManualSwitch  CurrentSetting=0
  Manual Switch1 : ManualSwitch  CurrentSetting=0
  Memory : Memory
  Mux : Mux  Inputs=2
  Plus : Sum
  Product : Product
  Subscribe : robotlib/Subscribe  topicSource=Select from ROS network  topic=/vehicle_acceleration_requested  messageType=std_msgs/Float64  sampleTime=-1  messageQueueLength=1
      settings: SourceProductBaseCode=RO
  Subscribe1 : robotlib/Subscribe  topicSource=Select from ROS network  topic=/TwistS  messageType=geometry_msgs/TwistStamped  sampleTime=-1  messageQueueLength=1
      settings: SourceProductBaseCode=RO
  Subscribe2 : robotlib/Subscribe  topicSource=Select from ROS network  topic=/steering_angle_command  messageType=std_msgs/Float64  sampleTime=-1  messageQueueLength=1
      settings: SourceProductBaseCode=RO
  Subtract1 : Sum  Inputs=+-
  Terminator_1 : Terminator
  Terminator_2 : Terminator
  Terminator_4 : Terminator
  acceleration_saturation : Subsystem
      mask Display: fprintf('Acceleration\nsaturation')
  acceleration_saturation1 : Subsystem
      mask Display: fprintf('Acceleration\nsaturation')
  Out1 : Outport
  Out2 : Outport  Port=2
  Out3 : Outport  Port=3
  Out4 : Outport  Port=4
  Out5 : Outport  Port=5
  Out6 : Outport  Port=6
  wires:
  Discrete-Time Integrator6/1 -> Out4/1
  Data Type Conversion8/1 -> Out3/1
  Discrete-Time Integrator4/1 -> Out6/1
  Data Type Conversion7/1 -> Out2/1
  Discrete-Time Integrator5/1 -> Out5/1
  Subscribe1/2 -> Bus Selector1/1
  Bus Selector1/3 -> Data Type Conversion8/1  "<Z>"
  Data Type Conversion9/1 -> Discrete-Time Integrator6/1
  Subscribe1/1 -> Terminator_4/1
  Data Type Conversion10/1 -> Discrete-Time Integrator5/1
  Bus Selector1/1 -> Data Type Conversion6/1  "<X>"
  Bus Selector1/4 -> Data Type Conversion9/1  "<X>"
  Bus Selector1/6 -> Data Type Conversion11/1  "<Z>"
  Bus Selector1/5 -> Data Type Conversion10/1  "<Y>"
  Bus Selector1/2 -> Data Type Conversion7/1  "<Y>"
  Data Type Conversion6/1 -> acceleration_saturation/2(In2)
  Manual Switch/1 -> Out1/1
  acceleration_saturation/1(Out1) -> Manual Switch/1
  acceleration_saturation1/1(Out1) -> Manual Switch/2
  Subscribe/2 -> Bus Selector2/1
  Subscribe/1 -> Terminator_2/1
  Bus Selector2/1 -> Data Type Conversion1/1  "<Data>"
  Plus/1 -> acceleration_saturation1/2(In2)
  Clock/1 -> Memory/1, Subtract1/1
  Memory/1 -> Subtract1/2
  Subtract1/1 -> Product/2
  Product/1 -> Plus/2
  Data Type Conversion11/1 -> Manual Switch1/1
  Mux/1 -> Fcn/1
  Data Type Conversion1/1 -> Product/1
  In1/1 -> Plus/1, Mux/2, acceleration_saturation1/1(In1), acceleration_saturation/1(In1)
  Fcn/1 -> Data Type Conversion2/1
  Data Type Conversion2/1 -> Manual Switch1/2
  Manual Switch1/1 -> Discrete-Time Integrator4/1
  Subscribe2/1 -> Terminator_1/1
  Data Type Conversion/1 -> Mux/1
  Bus Selector3/1 -> Data Type Conversion/1  "<Data>"
  Subscribe2/2 -> Bus Selector3/1

== system Simulation_cs_old/BMW_X5_SUV_1/SELF_Demux/compas converter ==
  rotz [rad] : Inport
  cart2compas : Subsystem
  rad2deg : Gain  Gain=180/pi
  heading [deg] : Outport
  wires:
  rad2deg/1 -> cart2compas/1(Angle [deg])
  rotz [rad]/1 -> rad2deg/1
  cart2compas/1(heading [deg]) -> heading [deg]/1

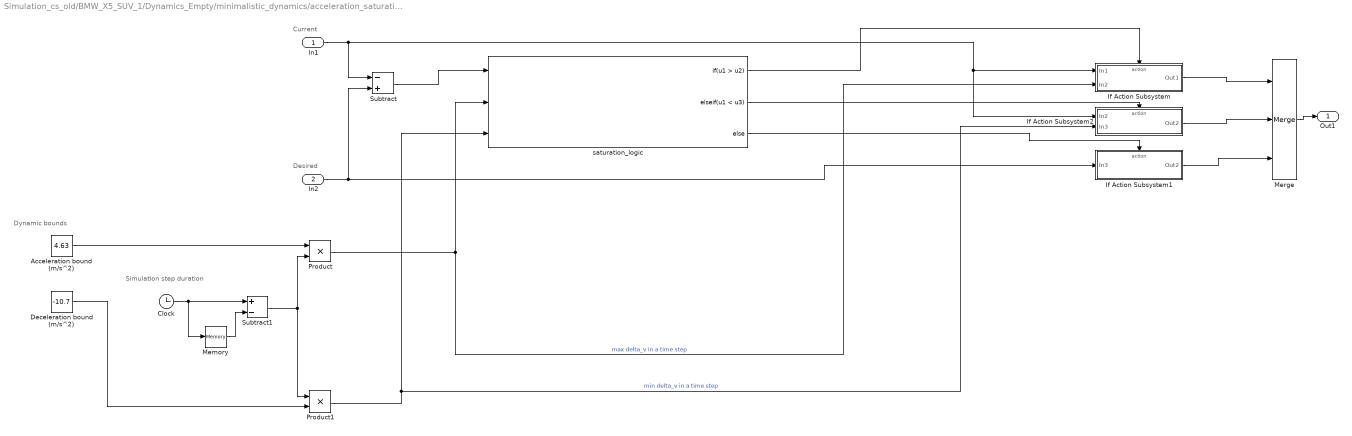
== system Simulation_cs_old/BMW_X5_SUV_1/Dynamics_Empty/minimalistic_dynamics/acceleration_saturation ==
  note: Desired
  note: Current
  note: Simulation step duration
  note: Dynamic bounds
  In1 : Inport
  In2 : Inport  Port=2
  Acceleration bound (m/s^2) : Constant  Value=4.63
  Clock : Clock
  Deceleration bound (m/s^2) : Constant  Value=-10.7
  If Action Subsystem : Subsystem  TreatAsAtomicUnit=on
      mask Display: fprintf('saturated acceleration\n')
  If Action Subsystem1 : Subsystem  TreatAsAtomicUnit=on
      mask Display: fprintf("desired passthrough")
  If Action Subsystem2 : Subsystem  TreatAsAtomicUnit=on
      mask Display: fprintf("saturated deceleration")
  Memory : Memory
  Merge : Merge  Inputs=3
  Product : Product
  Product1 : Product
  Subtract : Sum  Inputs=-+
  Subtract1 : Sum  Inputs=+-
  saturation_logic : If  NumInputs=3  IfExpression=u1 > u2  ElseIfExpressions=u1 < u3
      mask Display:
      | fprintf('Saturation\nLogic')
      | 
      | port_label('input',1,'desired_v - current_v')
      | port_label('input',2,'max delta_v allowed')
      | port_label('input',3,'min delta_v allowed')
      | port_label('output',1,'asking too much acceleration')
      | port_label('output',2,'asking too much deceleration')
      | port_label('output',3,'no saturation')
  Out1 : Outport
  wires:
  If Action Subsystem2/1(Out2) -> Merge/2
  If Action Subsystem1/1(Out2) -> Merge/3
  Product1/1 -> saturation_logic/3, If Action Subsystem2/2(In3)  "min delta_v in a time step"
  Acceleration bound (m/s^2)/1 -> Product/1
  Deceleration bound (m/s^2)/1 -> Product1/2
  If Action Subsystem/1(Out1) -> Merge/1
  saturation_logic/3 -> If Action Subsystem1/Action
  Merge/1 -> Out1/1
  saturation_logic/2 -> If Action Subsystem2/Action
  saturation_logic/1 -> If Action Subsystem/Action
  In1/1 -> If Action Subsystem/1(In1), If Action Subsystem2/1(In2), Subtract/1
  In2/1 -> If Action Subsystem1/1(In3), Subtract/2
  Subtract/1 -> saturation_logic/1
  Subtract1/1 -> Product1/1, Product/2
  Product/1 -> saturation_logic/2, If Action Subsystem/2(In2)  "max delta_v in a time step"
  Clock/1 -> Memory/1, Subtract1/1
  Memory/1 -> Subtract1/2

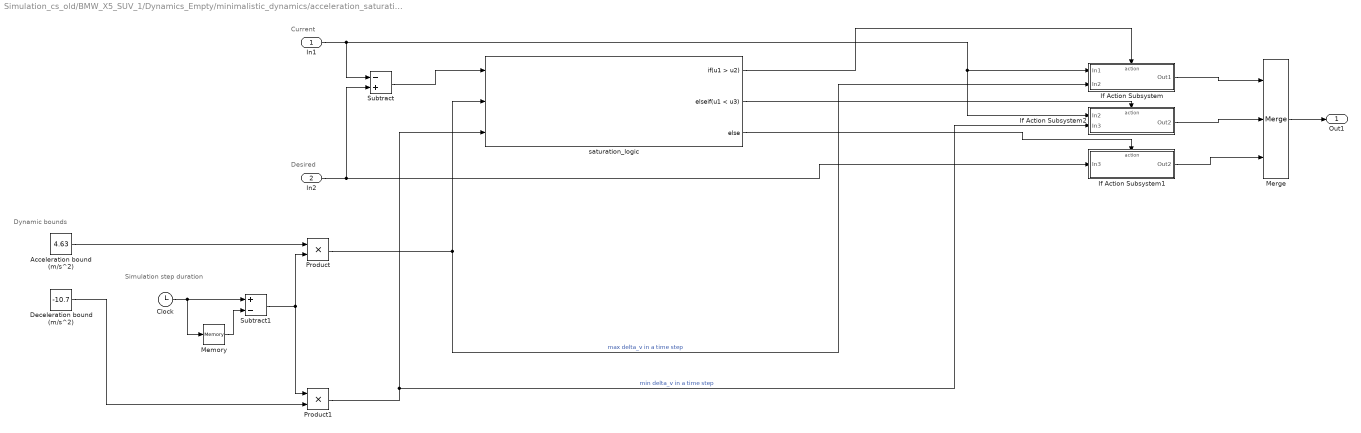
== system Simulation_cs_old/BMW_X5_SUV_1/Dynamics_Empty/minimalistic_dynamics/acceleration_saturation1 ==
  note: Desired
  note: Current
  note: Simulation step duration
  note: Dynamic bounds
  In1 : Inport
  In2 : Inport  Port=2
  Acceleration bound (m/s^2) : Constant  Value=4.63
  Clock : Clock
  Deceleration bound (m/s^2) : Constant  Value=-10.7
  If Action Subsystem : Subsystem  TreatAsAtomicUnit=on
      mask Display: fprintf('saturated acceleration\n')
  If Action Subsystem1 : Subsystem  TreatAsAtomicUnit=on
      mask Display: fprintf("desired passthrough")
  If Action Subsystem2 : Subsystem  TreatAsAtomicUnit=on
      mask Display: fprintf("saturated deceleration")
  Memory : Memory
  Merge : Merge  Inputs=3
  Product : Product
  Product1 : Product
  Subtract : Sum  Inputs=-+
  Subtract1 : Sum  Inputs=+-
  saturation_logic : If  NumInputs=3  IfExpression=u1 > u2  ElseIfExpressions=u1 < u3
      mask Display:
      | fprintf('Saturation\nLogic')
      | 
      | port_label('input',1,'desired_v - current_v')
      | port_label('input',2,'max delta_v allowed')
      | port_label('input',3,'min delta_v allowed')
      | port_label('output',1,'asking too much acceleration')
      | port_label('output',2,'asking too much deceleration')
      | port_label('output',3,'no saturation')
  Out1 : Outport
  wires:
  If Action Subsystem2/1(Out2) -> Merge/2
  If Action Subsystem1/1(Out2) -> Merge/3
  Product1/1 -> saturation_logic/3, If Action Subsystem2/2(In3)  "min delta_v in a time step"
  Acceleration bound (m/s^2)/1 -> Product/1
  Deceleration bound (m/s^2)/1 -> Product1/2
  If Action Subsystem/1(Out1) -> Merge/1
  saturation_logic/3 -> If Action Subsystem1/Action
  Merge/1 -> Out1/1
  saturation_logic/2 -> If Action Subsystem2/Action
  saturation_logic/1 -> If Action Subsystem/Action
  In1/1 -> If Action Subsystem/1(In1), If Action Subsystem2/1(In2), Subtract/1
  In2/1 -> If Action Subsystem1/1(In3), Subtract/2
  Subtract/1 -> saturation_logic/1
  Subtract1/1 -> Product1/1, Product/2
  Product/1 -> saturation_logic/2, If Action Subsystem/2(In2)  "max delta_v in a time step"
  Clock/1 -> Memory/1, Subtract1/1
  Memory/1 -> Subtract1/2

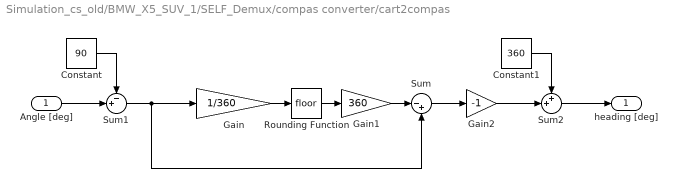
== system Simulation_cs_old/BMW_X5_SUV_1/SELF_Demux/compas converter/cart2compas ==
  Angle [deg] : Inport
  Constant : Constant  Value=90
  Constant1 : Constant  Value=360
  Gain : Gain  Gain=1/360
  Gain1 : Gain  Gain=360
  Gain2 : Gain  Gain=-1
  Rounding Function : Rounding
  Sum : Sum  Inputs=|-+
  Sum1 : Sum  Inputs=-+|
  Sum2 : Sum  Inputs=++|
  heading [deg] : Outport
  wires:
  Gain/1 -> Rounding Function/1
  Rounding Function/1 -> Gain1/1
  Gain1/1 -> Sum/1
  Angle [deg]/1 -> Sum1/2
  Sum/1 -> Gain2/1
  Sum1/1 -> Gain/1, Sum/2
  Constant/1 -> Sum1/1
  Gain2/1 -> Sum2/2
  Constant1/1 -> Sum2/1
  Sum2/1 -> heading [deg]/1

== system Simulation_cs_old/BMW_X5_SUV_1/Dynamics_Empty/minimalistic_dynamics/acceleration_saturation/If Action Subsystem ==
  In1 : Inport
  In2 : Inport  Port=2
  Action Port : ActionPort  ActionPortLabel=if(u1 > u2)
  Add : Sum
  Out1 : Outport
  wires:
  In2/1 -> Add/2
  In1/1 -> Add/1
  Add/1 -> Out1/1

== system Simulation_cs_old/BMW_X5_SUV_1/Dynamics_Empty/minimalistic_dynamics/acceleration_saturation/If Action Subsystem1 ==
  In3 : Inport
  Action Port : ActionPort  ActionPortLabel=else
  Out2 : Outport
  wires:
  In3/1 -> Out2/1

== system Simulation_cs_old/BMW_X5_SUV_1/Dynamics_Empty/minimalistic_dynamics/acceleration_saturation/If Action Subsystem2 ==
  In2 : Inport
  In3 : Inport  Port=2
  Action Port : ActionPort  ActionPortLabel=elseif(u1 < u3)
  Add : Sum
  Out2 : Outport
  wires:
  Add/1 -> Out2/1
  In3/1 -> Add/2
  In2/1 -> Add/1

== system Simulation_cs_old/BMW_X5_SUV_1/Dynamics_Empty/minimalistic_dynamics/acceleration_saturation1/If Action Subsystem ==
  In1 : Inport
  In2 : Inport  Port=2
  Action Port : ActionPort  ActionPortLabel=if(u1 > u2)
  Add : Sum
  Out1 : Outport
  wires:
  In2/1 -> Add/2
  In1/1 -> Add/1
  Add/1 -> Out1/1

== system Simulation_cs_old/BMW_X5_SUV_1/Dynamics_Empty/minimalistic_dynamics/acceleration_saturation1/If Action Subsystem1 ==
  In3 : Inport
  Action Port : ActionPort  ActionPortLabel=else
  Out2 : Outport
  wires:
  In3/1 -> Out2/1

== system Simulation_cs_old/BMW_X5_SUV_1/Dynamics_Empty/minimalistic_dynamics/acceleration_saturation1/If Action Subsystem2 ==
  In2 : Inport
  In3 : Inport  Port=2
  Action Port : ActionPort  ActionPortLabel=elseif(u1 < u3)
  Add : Sum
  Out2 : Outport
  wires:
  Add/1 -> Out2/1
  In3/1 -> Add/2
  In2/1 -> Add/1
